simulink model "powertrain_model"  (R2025a)
settings: Solver=ode23tb  StartTime=0.0  StopTime=simlength  FixedStep=tc  MaxStep=tc
values from neighbouring files (symbols this model uses):
  angle_error = angle_error_deg/180*pi    (= 0)    [init_model.m]
  CTRPIFF_CLIP_RELEASE = 0.001    [init_model.m]
  dead_time = dead_time_INV    (= 4.2e-07)    [init_model.m]
  dead_time_INV = 0.42e-6    (= 4.2e-07)    [init_model.m]
  DThs_init = 0    [init_model.m]
  emf_fb_p = 0.2    [init_model.m]
  emf_fb_p_ccaller_1 = emf_fb_p    (= 0.2)    [init_model.m]
  emf_fb_p_ccaller_2 = emf_fb_p    (= 0.2)    [init_model.m]
  emf_p = emf_fb_p*4/10    (= 0.08)    [init_model.m]
  emf_p_ccaller_1 = emf_fb_p_ccaller_1*4/10    (= 0.08)    [init_model.m]
  emf_p_ccaller_2 = emf_fb_p_ccaller_2*4/10    (= 0.08)    [init_model.m]
  fPWM_INV = 25e3    (= 25000)    [init_model.m]
  g0_reference_flt = fcut_reference_flt * ts_inv * 2*pi    (= 0.00100530964915)    [init_model.m]
  g1_reference_flt = 1 - g0_reference_flt    (= 0.998994690351)    [init_model.m]
  id_ref_if_pu = iload_rms_ref*sqrt(2)/ibez    [init_model.m]
  kalman_omega = kw    [init_model.m]
  kalman_theta = kg    [init_model.m]
  kg = K(1)    [init_model.m]
  ki_id = 2    [analysis_cc.m]    (also in init_model.m = 9)
  ki_iq = 9    [init_model.m]
  ki_w = 1    [init_model.m]
  kp_id = 0.15    [analysis_cc.m]    (also in init_model.m = 0.25)
  kp_iq = 0.2    [init_model.m]
  kp_w = 1    [init_model.m]
  kw = K(2)    [init_model.m]
  luenberger_l1 = Klo(1)    [init_model.m]
  luenberger_l2 = Klo(2)    [init_model.m]
  luenberger_l3 = Klo(3)    [init_model.m]
  motorc_m_scale = 2/3*Vdc_bez/ubez    [init_model.m]
  number_of_cells = 100    [init_model.m]
  omega_flt_fcut = 10    [init_model.m]
  omega_flt_g0 = omega_flt_fcut * ts_inv * 2*pi    (= 0.00251327412287)    [init_model.m]
  omega_flt_g1 = 1 - omega_flt_g0    (= 0.997486725877)    [init_model.m]
  omega_ref_if_pu = 1200*2*pi/omega_bez    [init_model.m]
  phase_compensation_omega = 0    [init_model.m]
  pwm_out_lim = 1    [init_model.m]
  Q = 10    [init_model.m]
  q1Kalman = ts_inv^2    (= 1.6e-09)    [init_model.m]
  q2Kalman = ts_inv^1    (= 4e-05)    [init_model.m]
  q3Kalman = 0    [init_model.m]
  rKalman = 1    [init_model.m]
  Tambient = 1    [init_model.m]
  tc = ts_inv/200    (= 2e-07)    [init_model.m]
  time_init = 0.025    [init_model.m]
  torque_ref = 64/ibez*torque_mode    [init_model.m]
  ts_inv = 1/fPWM_INV    (= 4e-05)    [init_model.m]
  tsample = ts_inv    (= 4e-05)    [init_model.m]
  u_flt_g0 = u_flt_fcut * ts_inv * 2*pi    (= 0.904778684234)    [init_model.m]
  u_flt_g1 = 1 - u_flt_g0    (= 0.0952213157661)    [init_model.m]
  Vdc_bez = 400    [init_model.m]
undefined symbols (not defined in the file or in its folder): b, ibez, Jm, Jm_norm, Ld_norm, Lq_norm, Ls_norm, magnitude, omega_bez, psi_bez, psi_m, psi_m_norm, R_RLload, Rload_eq, Rs_norm, tau_bez, weigth
libraries: fl_lib x100, nesl_utility x84, ee_lib x11, cstblocks x4, lithium_ion_cell_lib x1, simulink x1, pmsm_uvw_with_harmonics_lib x1, pmsm_spatial_harmonics_uvw_lib x1, flexshaft_lib x1
(part 1 of 6)
settings Model: SimulationMode=accelerator  Creator=dbagn  LastModifiedBy=dbagn
settings SolverCC: NumberNewtonIterations=3.0  ZeroCrossControl=DisableAll  AlgebraicLoopSolver=TrustRegion  SolverResetMethod=Robust
settings DataIOCC: SaveOutput=off  SignalLogging=off  DSMLogging=off  SaveTime=off  ReturnWorkspaceOutputs=off
settings OptimizationCC: ReuseModelBlockBuffer=off
settings DebuggingCC: UnconnectedInputMsg=warning  UnconnectedOutputMsg=warning  UnconnectedLineMsg=warning
settings ModelReferenceCC: EnableRefExpFcnMdlSchedulingChecks=on
settings SFSimCC: SimUserIncludeDirs=include  SimAnalyzeCustomCode=on
settings SFSimCC: SimCustomHeaderCode=|
  | #include "mavgflt.h"
  | #include "bemf_obsv.h"
  | #include "dqvector_pi.h"
  | #include "dqvector_pi_simulink.h"
  | #include "mavgflt_simulink.h"
  | #include "sv_pwm.h"
  | #include "bemf_obsv_simulink.h"
  | #include "bemf_obsv_load_est.h"
  | #include "bemf_obsv_load_est_simulink.h"
  | #include "sv_pwm_simulink.h"
  | #include "fb_state_machine.h"
  | #include "fb_state_machine_simulink.h"
settings SFSimCC: SimUserSources=|
  | dqvector_pi.c
  | dqvector_pi_simulink.c
  | mavgflt_simulink.c
  | mavgflt.c
  | bemf_obsv_simulink.c
  | bemf_obsv.c
  | bemf_obsv_load_est_simulink.c
  | bemf_obsv_load_est.c
  | sv_pwm.c
  | sv_pwm_simulink.c
  | fb_state_machine.c
  | fb_state_machine_simulink.c
settings RTWCC: GPUComputeCapability=3.5  DLArmComputeVersion=19.05

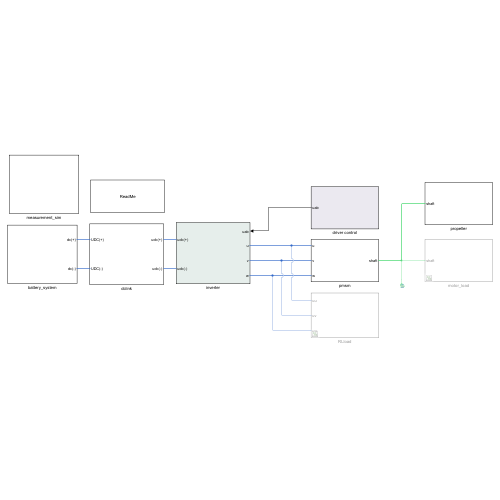
[thumbnail: Simulink's stored preview of the top-level diagram]
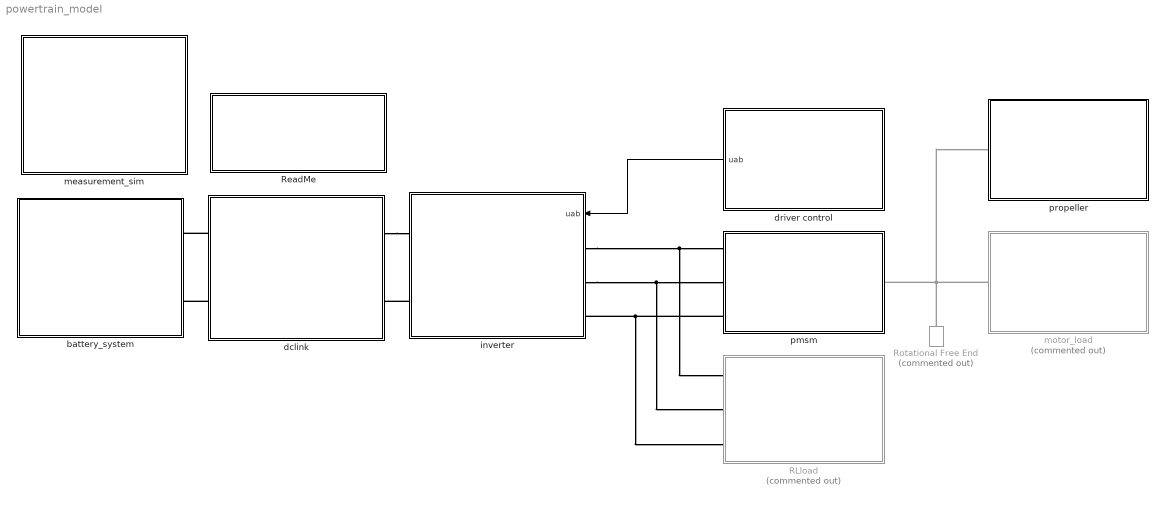
== system powertrain_model ==
  RLload : Subsystem  Commented=on
  ReadMe : Subsystem
      mask Display: disp('ReadMe')
  Rotational Free End : fl_lib/Mechanical/Rotational Elements/Rotational Free End  Commented=on  w_specify=off  w_priority=None  w=0 rad/s  w_nominal_specify=off  w_nominal_value=1  w_nominal_unit=rad/s
  battery_system : Subsystem
  dclink : Subsystem
  driver control : Subsystem
  inverter : Subsystem
  measurement_sim : Subsystem
  motor_load : Subsystem  Commented=on
  pmsm : Subsystem
  propeller : Subsystem
  wires:
  driver control/1(uab) -> inverter/1(uab)
  connections:
  dclink/LConn1 -- battery_system/RConn1
  dclink/LConn2 -- battery_system/RConn2
  inverter/RConn2 -- dclink/RConn2
  dclink/RConn1 -- inverter/RConn1
  motor_load/RConn1 -- pmsm/RConn1 -- propeller/LConn1 -- Rotational Free End/LConn1
  pmsm/LConn3 -- RLload/LConn3 -- inverter/LConn3
  inverter/LConn2 -- RLload/LConn2 -- pmsm/LConn2
  inverter/LConn1 -- RLload/LConn1 -- pmsm/LConn1

== system powertrain_model/RLload ==
  Bus Creator1 : BusCreator  Inputs=3
  Current Sensor : fl_lib/Electrical/Electrical Sensors/Current Sensor
  Current Sensor1 : fl_lib/Electrical/Electrical Sensors/Current Sensor
  Current Sensor2 : fl_lib/Electrical/Electrical Sensors/Current Sensor
  Inductor : ee_lib/Passive/Inductor  l=L_RLload H  enable_L_tol=0  L_tol=20  tol_distribution=1  nSigma=4  r=0 Ohm  g=1e-9 1/Ohm  enable_operating_limits=0  operating_limit_action=2  max_working_current=1 A  power_rating=1 W  i_L_specify=off  i_L_priority=High  i_L=0 A  i_L_nominal_specify=off  i_L_nominal_value=1  i_L_nominal_unit=A
  Inductor1 : ee_lib/Passive/Inductor  l=L_RLload H  enable_L_tol=0  L_tol=20  tol_distribution=1  nSigma=4  r=0 Ohm  g=1e-9 1/Ohm  enable_operating_limits=0  operating_limit_action=2  max_working_current=1 A  power_rating=1 W  i_L_specify=off  i_L_priority=High  i_L=0 A  i_L_nominal_specify=off  i_L_nominal_value=1  i_L_nominal_unit=A
  Inductor2 : ee_lib/Passive/Inductor  l=L_RLload H  enable_L_tol=0  L_tol=20  tol_distribution=1  nSigma=4  r=0 Ohm  g=1e-9 1/Ohm  enable_operating_limits=0  operating_limit_action=2  max_working_current=1 A  power_rating=1 W  i_L_specify=off  i_L_priority=High  i_L=0 A  i_L_nominal_specify=off  i_L_nominal_value=1  i_L_nominal_unit=A
  PS-Simulink Converter1 : nesl_utility/PS-Simulink Converter  PhysicalDomain=network_engine_domain  SubClassName=ps_output  LeftPortType=input  RightPortType=output  PseudoPeriodic=off  Frequencies=[]  VectorFormat=1-D array  Unit=A  AffineConversion=off
  PS-Simulink Converter2 : nesl_utility/PS-Simulink Converter  PhysicalDomain=network_engine_domain  SubClassName=ps_output  LeftPortType=input  RightPortType=output  PseudoPeriodic=off  Frequencies=[]  VectorFormat=1-D array  Unit=A  AffineConversion=off
  PS-Simulink Converter3 : nesl_utility/PS-Simulink Converter  PhysicalDomain=network_engine_domain  SubClassName=ps_output  LeftPortType=input  RightPortType=output  PseudoPeriodic=off  Frequencies=[]  VectorFormat=1-D array  Unit=A  AffineConversion=off
  Resistor : fl_lib/Electrical/Electrical Elements/Resistor  R=R_RLload Ohm  i_specify=off  i_priority=None  i=0 A  i_nominal_specify=off  i_nominal_value=1  i_nominal_unit=A  v_specify=off  v_priority=None  v=0 V  v_nominal_specify=off  v_nominal_value=1  v_nominal_unit=V
  Resistor1 : fl_lib/Electrical/Electrical Elements/Resistor  R=R_RLload Ohm  i_specify=off  i_priority=None  i=0 A  i_nominal_specify=off  i_nominal_value=1  i_nominal_unit=A  v_specify=off  v_priority=None  v=0 V  v_nominal_specify=off  v_nominal_value=1  v_nominal_unit=V
  Resistor2 : fl_lib/Electrical/Electrical Elements/Resistor  R=R_RLload Ohm  i_specify=off  i_priority=None  i=0 A  i_nominal_specify=off  i_nominal_value=1  i_nominal_unit=A  v_specify=off  v_priority=None  v=0 V  v_nominal_specify=off  v_nominal_value=1  v_nominal_unit=V
  iuvw_load : Scope
      settings: SampleTime=tc  ActiveDisplayYMinimum=-116.88009  ActiveDisplayYMaximum=116.86904
  uu : PMIOPort  Side=Left
  uv : PMIOPort  Port=2  Side=Left
  uw : PMIOPort  Port=3  Side=Left
  wires:
  PS-Simulink Converter1/1 -> Bus Creator1/1  "iu_load_sim"
  Bus Creator1/1 -> iuvw_load/1
  PS-Simulink Converter3/1 -> Bus Creator1/3  "iw_load_sim"
  PS-Simulink Converter2/1 -> Bus Creator1/2  "iv_load_sim"
  connections:
  Resistor1/LConn1 -- uv/RConn1
  uu/RConn1 -- Resistor/LConn1
  Resistor2/LConn1 -- uw/RConn1
  Inductor1/LConn1 -- Resistor1/RConn1
  Resistor/RConn1 -- Inductor/LConn1
  Inductor2/LConn1 -- Resistor2/RConn1
  PS-Simulink Converter3/LConn1 -- Current Sensor2/RConn1
  Current Sensor1/RConn1 -- PS-Simulink Converter2/LConn1
  Current Sensor/RConn2 -- Current Sensor2/RConn2 -- Current Sensor1/RConn2
  Current Sensor/RConn1 -- PS-Simulink Converter1/LConn1
  Current Sensor/LConn1 -- Inductor/RConn1
  Inductor2/RConn1 -- Current Sensor2/LConn1
  Inductor1/RConn1 -- Current Sensor1/LConn1

== system powertrain_model/ReadMe ==

== system powertrain_model/battery_system ==
  DC Voltage Source : fl_lib/Electrical/Electrical Sources/DC Voltage Source  Commented=on  v0=Vdc_bez V
  Electrical Reference2 : fl_lib/Electrical/Electrical Elements/Electrical Reference
  Solver Configuration : nesl_utility/Solver Configuration  PhysicalDomain=network_engine_domain  SubClassName=solver  LeftPortType=input  RightPortType=generic  Tones=[]  Harmonics=[]  SimulateNoise=off  Profile=off  UseLocalSampling=off  EnableSwitchedLinearOptims=on  FrequencyDomain=off  UseCCode=off  RelTol=0.001  AbsTol=0.001  MinStep=1e-09  ToWorkspace=off  RevertToSquareIcSolve=off  NumHomotopyIterations=100  PhasorMode=off  PhasorModeNumHarmonics=1  ConsistencySolver=NEWTON_FTOL  IndexReductionMethod=DerivativeReplacement  DoDC=off  ResidualTolerance=1e-09  ConsistencyTolSource=GLOBAL  ConsistencyAbsTol=0.001  ConsistencyRelTol=0.001  ConsistencyTolFactor=0.001  UseLocalSolver=on  LocalSolverChoice=NE_BACKWARD_EULER_ADVANCER  ResolveIndetEquations=on  FunctionEvalNumThread=1  LocalSolverSampleTime=tc  DoFixedCost=on  MaxNonlinIter=5  MaxModeIter=2  ComputeImpulses=off  ImpulseIterations=2  LinearAlgebra=auto  LinearAlgebraNumThread=0  EquationFormulation=NE_TIME_EF  DelaysMemoryBudget=1024  AutomaticFiltering=on  FilteringTimeConstant=0.001  PartitionStorageMethod=AS_NEEDED  PartitionMemoryBudget=1024  PartitionMethod=ROBUST  MultibodyUseLocalSolver=off  MultibodyLocalSolverChoice=ODE1  MultibodyLocalSolverSampleTime=0.001
  battery_system : Subsystem
  dc(+) : PMIOPort  Side=Right
  dc(-) : PMIOPort  Port=2  Side=Right
  connections:
  Solver Configuration/RConn1 -- DC Voltage Source/RConn1 -- Electrical Reference2/LConn1 -- dc(-)/RConn1
  DC Voltage Source/LConn1 -- dc(+)/RConn1 -- battery_system/RConn1

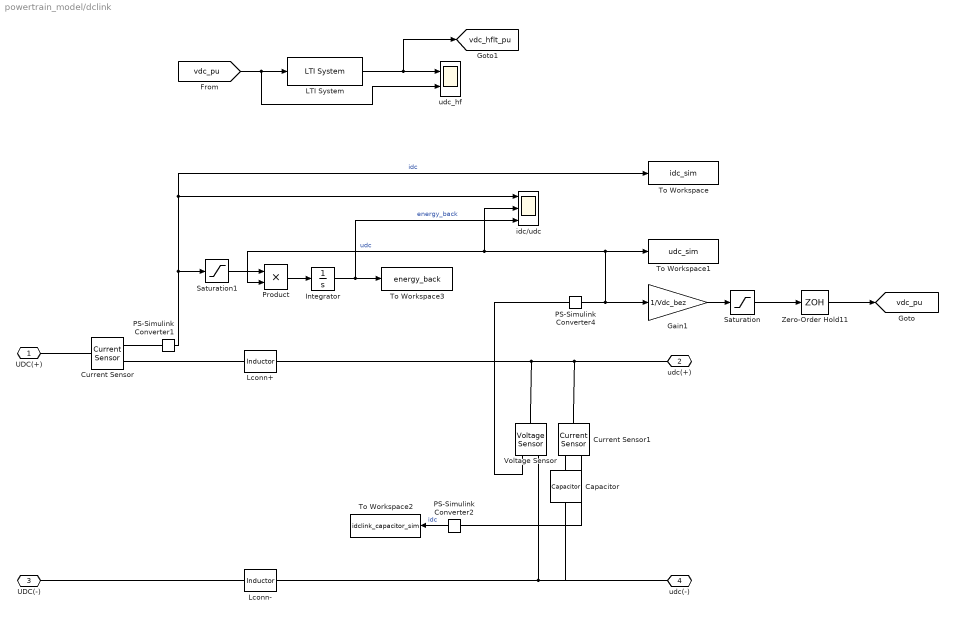
== system powertrain_model/dclink ==
  Capacitor : fl_lib/Electrical/Electrical Elements/Capacitor  c=CFi F  r=1e-3 Ohm  g=0 1/Ohm  i_specify=off  i_priority=None  i=0 A  i_nominal_specify=off  i_nominal_value=1  i_nominal_unit=A  v_specify=off  v_priority=None  v=Vdc_bez V  v_nominal_specify=off  v_nominal_value=1  v_nominal_unit=V  vc_specify=on  vc_priority=High  vc=Vdc V  vc_nominal_specify=off  vc_nominal_value=1  vc_nominal_unit=V
  Current Sensor : fl_lib/Electrical/Electrical Sensors/Current Sensor
  Current Sensor1 : fl_lib/Electrical/Electrical Sensors/Current Sensor
  Gain1 : Gain  Gain=1/Vdc_bez
  Integrator : Integrator
  LTI System : cstblocks/LTI System  sys=hpf2q_d  IC=[]  PadeOrder=0
  Lconn+ : fl_lib/Electrical/Electrical Elements/Inductor  l=0.5e-6 H  r=5e-3 Ohm  g=1e-9 1/Ohm  i_specify=on  i_priority=High  i=0 A  i_nominal_specify=off  i_nominal_value=1  i_nominal_unit=A  v_specify=off  v_priority=None  v=0 V  v_nominal_specify=off  v_nominal_value=1  v_nominal_unit=V  i_L_specify=off  i_L_priority=High  i_L=0 A  i_L_nominal_specify=off  i_L_nominal_value=1  i_L_nominal_unit=A
  Lconn- : fl_lib/Electrical/Electrical Elements/Inductor  l=0.5e-6 H  r=5e-3 Ohm  g=1e-9 1/Ohm  i_specify=on  i_priority=High  i=0 A  i_nominal_specify=off  i_nominal_value=1  i_nominal_unit=A  v_specify=off  v_priority=None  v=0 V  v_nominal_specify=off  v_nominal_value=1  v_nominal_unit=V  i_L_specify=off  i_L_priority=High  i_L=0 A  i_L_nominal_specify=off  i_L_nominal_value=1  i_L_nominal_unit=A
  PS-Simulink Converter1 : nesl_utility/PS-Simulink Converter  PhysicalDomain=network_engine_domain  SubClassName=ps_output  LeftPortType=input  RightPortType=output  PseudoPeriodic=off  Frequencies=[]  VectorFormat=1-D array  Unit=A  AffineConversion=on
  PS-Simulink Converter2 : nesl_utility/PS-Simulink Converter  PhysicalDomain=network_engine_domain  SubClassName=ps_output  LeftPortType=input  RightPortType=output  PseudoPeriodic=off  Frequencies=[]  VectorFormat=1-D array  Unit=A  AffineConversion=on
  PS-Simulink Converter4 : nesl_utility/PS-Simulink Converter  PhysicalDomain=network_engine_domain  SubClassName=ps_output  LeftPortType=input  RightPortType=output  PseudoPeriodic=off  Frequencies=[]  VectorFormat=1-D array  Unit=V  AffineConversion=on
  Product : Product
  Saturation : Saturate  UpperLimit=inf  LowerLimit=0.1
  Saturation1 : Saturate  UpperLimit=0  LowerLimit=-inf
  To Workspace : ToWorkspace  VariableName=idc_sim  SampleTime=tc
      settings: MaxDataPoints=Nc
  To Workspace1 : ToWorkspace  VariableName=udc_sim  SampleTime=tc
      settings: MaxDataPoints=Nc
  To Workspace2 : ToWorkspace  VariableName=idclink_capacitor_sim  SampleTime=tc
      settings: MaxDataPoints=Nc
  To Workspace3 : ToWorkspace  VariableName=energy_back  SampleTime=tc
      settings: MaxDataPoints=Nc
  Voltage Sensor : fl_lib/Electrical/Electrical Sensors/Voltage Sensor
  Zero-Order Hold11 : ZeroOrderHold  SampleTime=ts_inv
  idc/udc : Scope  NumInputPorts=3
      settings: SampleTime=tc  ActiveDisplayYMinimum=-8.28263  ActiveDisplayYMaximum=4.59214
  udc_hf : Scope  NumInputPorts=2
      settings: SampleTime=ts_inv  ActiveDisplayYMinimum=-0.00098  ActiveDisplayYMaximum=0.00078
  UDC(+) : PMIOPort  Side=Left
  udc(+) : PMIOPort  Port=2  Side=Right
  UDC(-) : PMIOPort  Port=3  Side=Left
  udc(-) : PMIOPort  Port=4  Side=Right
  tag scope: vdc_hflt_pu=global, vdc_pu=global
  wires:
  Saturation/1 -> Zero-Order Hold11/1
  PS-Simulink Converter4/1 -> idc/udc/2, Product/2, To Workspace1/1, Gain1/1  "udc"
  Gain1/1 -> Saturation/1
  PS-Simulink Converter1/1 -> Saturation1/1, To Workspace/1, idc/udc/1  "idc"
  PS-Simulink Converter2/1 -> To Workspace2/1  "idc"
  Saturation1/1 -> Product/1
  Product/1 -> Integrator/1
  Integrator/1 -> idc/udc/3, To Workspace3/1  "energy_back"
  LTI System/1 -> [vdc_hflt_pu], udc_hf/1
  [vdc_pu] -> udc_hf/2, LTI System/1
  Zero-Order Hold11/1 -> [vdc_pu]
  connections:
  PS-Simulink Converter4/LConn1 -- Voltage Sensor/RConn1
  Current Sensor1/RConn1 -- PS-Simulink Converter2/LConn1
  PS-Simulink Converter1/LConn1 -- Current Sensor/RConn1
  Current Sensor/RConn2 -- Lconn+/LConn1
  Current Sensor/LConn1 -- UDC(+)/RConn1
  Current Sensor1/RConn2 -- Capacitor/LConn1
  Lconn-/RConn1 -- UDC(-)/RConn1
  Lconn+/RConn1 -- Voltage Sensor/LConn1 -- Current Sensor1/LConn1 -- udc(+)/RConn1
  Voltage Sensor/RConn2 -- Lconn-/LConn1 -- Capacitor/RConn1 -- udc(-)/RConn1

== system powertrain_model/driver control ==
  Mux : Mux  Inputs=2
  Mux1 : Mux  Inputs=2
  Mux2 : Mux  Inputs=2
  Sum1 : Sum  Inputs=+++
  Sum2 : Sum  Inputs=+++
  bemf_observer : Subsystem
  current_ctrl : Subsystem
  i/f references : Subsystem  Commented=on
  id/iq/torque/omega : Scope  NumInputPorts=3
      settings: SampleTime=ts_inv  ActiveDisplayYMinimum=-0.27921550957244479  ActiveDisplayYMaximum=1.2654943086208228  DataLoggingVariableName=ScopeData3
  normalization1 : Gain  Gain=1/tau_bez
  normalization2 : Gain  Gain=1/omega_bez
  speed_loop : Subsystem  Commented=on
  torque_reference_generator : Subsystem
  uab : Outport  VectorParamsAs1DForOutWhenUnconnected=off
  wires:
  Mux/1 -> id/iq/torque/omega/1
  [torque_pmsm] -> normalization1/1
  current_ctrl/1(uab) -> uab/1  "uab"
  Sum2/1 -> current_ctrl/2(iq_ref)  "iq_ref"
  normalization1/1 -> Mux1/1  "torque"
  [iq_inverter_pu] -> Mux/2  "iq_inverter_pu"
  [id_inverter_pu] -> Mux/1  "id_inverter_pu"
  [omega_pmsm] -> normalization2/1  "omega_pmsm"
  normalization2/1 -> Mux1/2  "omega_pmsm"
  Mux1/1 -> id/iq/torque/omega/2
  [omega_pu_hat_flt] -> Mux2/1  "omega_hat_flt"
  [omega_pu_hat] -> Mux2/2  "omega_hat"
  Mux2/1 -> id/iq/torque/omega/3
  Sum1/1 -> current_ctrl/1(id_ref)  "iq_ref"
  i/f references/1(id_if_pu) -> Sum1/2
  torque_reference_generator/1(iq_ref) -> Sum2/3  "torque_ref_pu"
  torque_reference_generator/2(id_ref) -> Sum1/3
  i/f references/2(iq_if_pu) -> Sum2/2
  speed_loop/2(id_ref) -> Sum1/1
  speed_loop/1(iq_ref) -> Sum2/1  "torque_ref_pu"

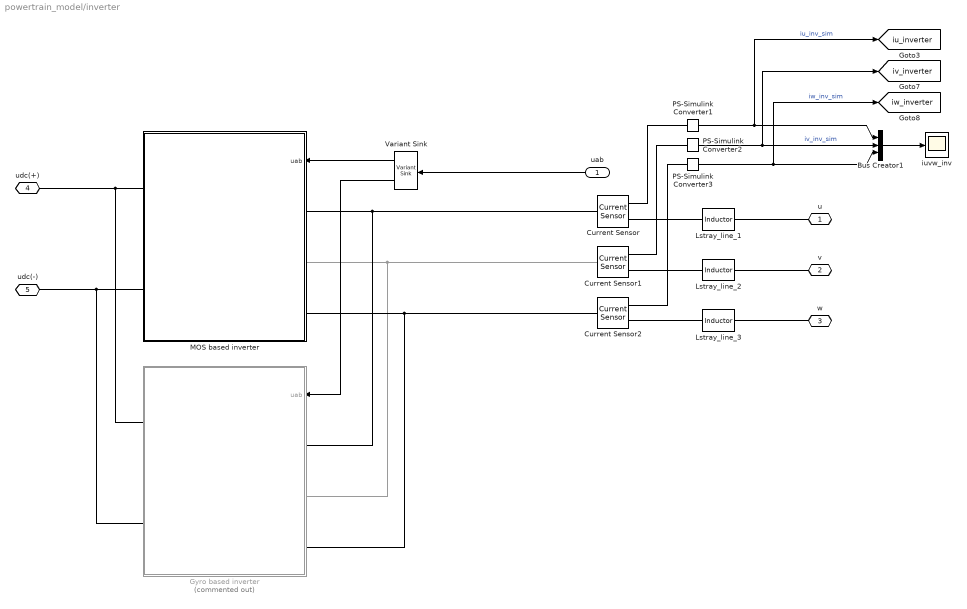
== system powertrain_model/inverter ==
  uab : Inport
  Bus Creator1 : BusCreator  Inputs=3
  Current Sensor : fl_lib/Electrical/Electrical Sensors/Current Sensor
  Current Sensor1 : fl_lib/Electrical/Electrical Sensors/Current Sensor
  Current Sensor2 : fl_lib/Electrical/Electrical Sensors/Current Sensor
  Gyro based inverter : Subsystem  Commented=on
  Lstray_line_1 : ee_lib/Passive/Inductor  l=5e-6 H  enable_L_tol=ee.enum.toleranceApplication.none  L_tol=20  tol_distribution=ee.enum.toleranceDistribution.uniform  nSigma=4  r=0 Ohm  g=1e-9 1/Ohm  enable_operating_limits=ee.enum.enable.no  operating_limit_action=ee.enum.passive.reportOpLim.warn  max_working_current=1 A  power_rating=1 W  i_L_specify=on  i_L_priority=High  i_L=0 A  i_L_nominal_specify=off  i_L_nominal_value=1  i_L_nominal_unit=A
  Lstray_line_2 : ee_lib/Passive/Inductor  l=5e-6 H  enable_L_tol=ee.enum.toleranceApplication.none  L_tol=20  tol_distribution=ee.enum.toleranceDistribution.uniform  nSigma=4  r=0 Ohm  g=1e-9 1/Ohm  enable_operating_limits=ee.enum.enable.no  operating_limit_action=ee.enum.passive.reportOpLim.warn  max_working_current=1 A  power_rating=1 W  i_L_specify=on  i_L_priority=High  i_L=0 A  i_L_nominal_specify=off  i_L_nominal_value=1  i_L_nominal_unit=A
  Lstray_line_3 : ee_lib/Passive/Inductor  l=5e-6 H  enable_L_tol=ee.enum.toleranceApplication.none  L_tol=20  tol_distribution=ee.enum.toleranceDistribution.uniform  nSigma=4  r=0 Ohm  g=1e-9 1/Ohm  enable_operating_limits=ee.enum.enable.no  operating_limit_action=ee.enum.passive.reportOpLim.warn  max_working_current=1 A  power_rating=1 W  i_L_specify=on  i_L_priority=High  i_L=0 A  i_L_nominal_specify=off  i_L_nominal_value=1  i_L_nominal_unit=A
  MOS based inverter : Subsystem
  PS-Simulink Converter1 : nesl_utility/PS-Simulink Converter  PhysicalDomain=network_engine_domain  SubClassName=ps_output  LeftPortType=input  RightPortType=output  PseudoPeriodic=off  Frequencies=[]  VectorFormat=1-D array  Unit=A  AffineConversion=off
  PS-Simulink Converter2 : nesl_utility/PS-Simulink Converter  PhysicalDomain=network_engine_domain  SubClassName=ps_output  LeftPortType=input  RightPortType=output  PseudoPeriodic=off  Frequencies=[]  VectorFormat=1-D array  Unit=A  AffineConversion=off
  PS-Simulink Converter3 : nesl_utility/PS-Simulink Converter  PhysicalDomain=network_engine_domain  SubClassName=ps_output  LeftPortType=input  RightPortType=output  PseudoPeriodic=off  Frequencies=[]  VectorFormat=1-D array  Unit=A  AffineConversion=off
  Variant Sink : VariantSink  VariantControls={use_gyro_model == 0, use_gyro_model == 1}
      settings: AllowZeroVariantControls=on
  iuvw_inv : Scope
      settings: SampleTime=tc  ActiveDisplayYMinimum=-190.27982  ActiveDisplayYMaximum=181.88216
  u : PMIOPort  Side=Left
  v : PMIOPort  Port=2  Side=Left
  w : PMIOPort  Port=3  Side=Left
  udc(+) : PMIOPort  Port=4  Side=Right
  udc(-) : PMIOPort  Port=5  Side=Right
  tag scope: iu_inverter=global, iv_inverter=global, iw_inverter=global
  wires:
  Bus Creator1/1 -> iuvw_inv/1
  PS-Simulink Converter3/1 -> [iw_inverter], Bus Creator1/3  "iw_inv_sim"
  PS-Simulink Converter1/1 -> [iu_inverter], Bus Creator1/1  "iu_inv_sim"
  PS-Simulink Converter2/1 -> [iv_inverter], Bus Creator1/2  "iv_inv_sim"
  uab/1 -> Variant Sink/1
  Variant Sink/1 -> MOS based inverter/1(uab)
  Variant Sink/2 -> Gyro based inverter/1(uab)
  connections:
  Gyro based inverter/LConn2 -- MOS based inverter/LConn2 -- Current Sensor1/LConn1
  MOS based inverter/LConn1 -- Current Sensor/LConn1 -- Gyro based inverter/LConn1
  MOS based inverter/LConn3 -- Current Sensor2/LConn1 -- Gyro based inverter/LConn3
  udc(+)/RConn1 -- Gyro based inverter/RConn1 -- MOS based inverter/RConn1
  udc(-)/RConn1 -- Gyro based inverter/RConn2 -- MOS based inverter/RConn2
  Lstray_line_3/RConn1 -- w/RConn1
  PS-Simulink Converter3/LConn1 -- Current Sensor2/RConn1
  Current Sensor1/RConn1 -- PS-Simulink Converter2/LConn1
  Current Sensor1/RConn2 -- Lstray_line_2/LConn1
  Current Sensor/RConn1 -- PS-Simulink Converter1/LConn1
  Current Sensor/RConn2 -- Lstray_line_1/LConn1
  Lstray_line_2/RConn1 -- v/RConn1
  Current Sensor2/RConn2 -- Lstray_line_3/LConn1
  u/RConn1 -- Lstray_line_1/RConn1

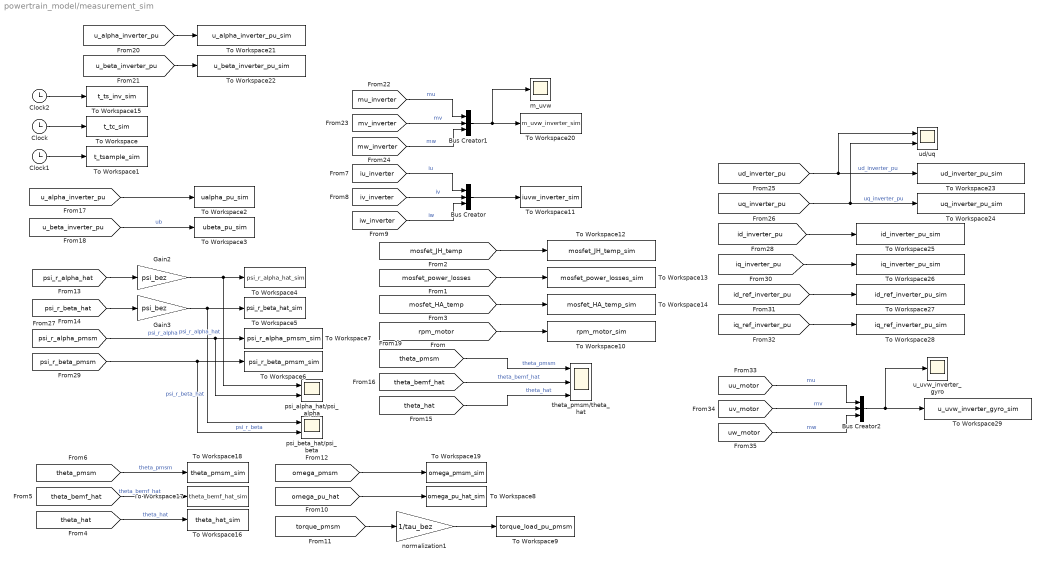
== system powertrain_model/measurement_sim ==
  Bus Creator : BusCreator  Inputs=3
  Bus Creator1 : BusCreator  Inputs=3
  Bus Creator2 : BusCreator  Inputs=3
  Clock : Clock
  Clock1 : Clock
  Clock2 : Clock
  Gain2 : Gain  Gain=psi_bez
  Gain3 : Gain  Gain=psi_bez
  To Workspace : ToWorkspace  VariableName=t_tc_sim  SampleTime=tc
      settings: MaxDataPoints=Nc
  To Workspace1 : ToWorkspace  VariableName=t_tsample_sim  SampleTime=tsample
      settings: MaxDataPoints=Nsample
  To Workspace10 : ToWorkspace  VariableName=rpm_motor_sim  SampleTime=ts_inv
      settings: MaxDataPoints=Ns_inv
  To Workspace11 : ToWorkspace  VariableName=iuvw_inverter_sim  SampleTime=tc
      settings: MaxDataPoints=Nc
  To Workspace12 : ToWorkspace  VariableName=mosfet_JH_temp_sim  SampleTime=tc
      settings: MaxDataPoints=Nc
  To Workspace13 : ToWorkspace  VariableName=mosfet_power_losses_sim  SampleTime=tc
      settings: MaxDataPoints=Nc
  To Workspace14 : ToWorkspace  VariableName=mosfet_HA_temp_sim  SampleTime=tc
      settings: MaxDataPoints=Nc
  To Workspace15 : ToWorkspace  VariableName=t_ts_inv_sim  SampleTime=ts_inv
      settings: MaxDataPoints=Ns_inv
  To Workspace16 : ToWorkspace  VariableName=theta_hat_sim  SampleTime=ts_inv
      settings: MaxDataPoints=Ns_inv
  To Workspace17 : ToWorkspace  VariableName=theta_bemf_hat_sim  SampleTime=ts_inv
      settings: MaxDataPoints=Ns_inv
  To Workspace18 : ToWorkspace  VariableName=theta_pmsm_sim  SampleTime=ts_inv
      settings: MaxDataPoints=Ns_inv
  To Workspace19 : ToWorkspace  VariableName=omega_pmsm_sim  SampleTime=ts_inv
      settings: MaxDataPoints=Ns_inv
  To Workspace2 : ToWorkspace  VariableName=ualpha_pu_sim  SampleTime=ts_inv
      settings: MaxDataPoints=Ns_inv
  To Workspace20 : ToWorkspace  VariableName=m_uvw_inverter_sim  SampleTime=tc
      settings: MaxDataPoints=Nc
  To Workspace21 : ToWorkspace  VariableName=u_alpha_inverter_pu_sim  SampleTime=tc
      settings: MaxDataPoints=Nc
  To Workspace22 : ToWorkspace  VariableName=u_beta_inverter_pu_sim  SampleTime=tc
      settings: MaxDataPoints=Nc
  To Workspace23 : ToWorkspace  VariableName=ud_inverter_pu_sim  SampleTime=tc
      settings: MaxDataPoints=Nc
  To Workspace24 : ToWorkspace  VariableName=uq_inverter_pu_sim  SampleTime=tc
      settings: MaxDataPoints=Nc
  To Workspace25 : ToWorkspace  VariableName=id_inverter_pu_sim  SampleTime=tc
      settings: MaxDataPoints=Nc
  To Workspace26 : ToWorkspace  VariableName=iq_inverter_pu_sim  SampleTime=tc
      settings: MaxDataPoints=Nc
  To Workspace27 : ToWorkspace  VariableName=id_ref_inverter_pu_sim  SampleTime=tc
      settings: MaxDataPoints=Nc
  To Workspace28 : ToWorkspace  VariableName=iq_ref_inverter_pu_sim  SampleTime=tc
      settings: MaxDataPoints=Nc
  To Workspace29 : ToWorkspace  VariableName=u_uvw_inverter_gyro_sim  SampleTime=tc
      settings: MaxDataPoints=Nc
  To Workspace3 : ToWorkspace  VariableName=ubeta_pu_sim  SampleTime=ts_inv
      settings: MaxDataPoints=Ns_inv
  To Workspace4 : ToWorkspace  VariableName=psi_r_alpha_hat_sim  SampleTime=ts_inv
      settings: MaxDataPoints=Ns_inv
  To Workspace5 : ToWorkspace  VariableName=psi_r_beta_hat_sim  SampleTime=ts_inv
      settings: MaxDataPoints=Ns_inv
  To Workspace6 : ToWorkspace  VariableName=psi_r_beta_pmsm_sim  SampleTime=ts_inv
      settings: MaxDataPoints=Ns_inv
  To Workspace7 : ToWorkspace  VariableName=psi_r_alpha_pmsm_sim  SampleTime=ts_inv
      settings: MaxDataPoints=Ns_inv
  To Workspace8 : ToWorkspace  VariableName=omega_pu_hat_sim  SampleTime=ts_inv
      settings: MaxDataPoints=Ns_inv
  To Workspace9 : ToWorkspace  VariableName=torque_load_pu_pmsm  SampleTime=ts_inv
      settings: MaxDataPoints=Ns_inv
  m_uvw : Scope
      settings: SampleTime=ts_inv  ActiveDisplayYMinimum=0.41574  ActiveDisplayYMaximum=0.59549  DataLoggingVariableName=ScopeData2
  normalization1 : Gain  Gain=1/tau_bez
  psi_alpha_hat/psi_alpha : Scope  NumInputPorts=2
      settings: SampleTime=ts_inv  ActiveDisplayYMinimum=-0.030406717651633802  ActiveDisplayYMaximum=0.030440385944099833  DataLoggingVariableName=ScopeData2
  psi_beta_hat/psi_beta : Scope  NumInputPorts=2
      settings: SampleTime=ts_inv  ActiveDisplayYMinimum=-0.02688  ActiveDisplayYMaximum=0.02688  DataLoggingVariableName=ScopeData3
  theta_pmsm/theta_hat : Scope  NumInputPorts=3
      settings: SampleTime=tc  ActiveDisplayYMinimum=-3.9269753976279205  ActiveDisplayYMaximum=3.9268824807461784
  u_uvw_inverter_gyro : Scope
      settings: SampleTime=ts_inv  ActiveDisplayYMinimum=-1.24968  ActiveDisplayYMaximum=1.24993
  ud/uq : Scope  NumInputPorts=2
      settings: SampleTime=ts_inv  ActiveDisplayYMinimum=-0.81271  ActiveDisplayYMaximum=0.72345
  wires:
  [psi_r_beta_hat] -> Gain3/1
  [psi_r_alpha_hat] -> Gain2/1
  [u_alpha_inverter_pu] -> To Workspace2/1
  [psi_r_alpha_pmsm] -> psi_alpha_hat/psi_alpha/2, To Workspace7/1  "psi_r_alpha"
  Clock1/1 -> To Workspace1/1
  Clock/1 -> To Workspace/1
  [u_beta_inverter_pu] -> To Workspace3/1  "ub"
  [psi_r_beta_pmsm] -> To Workspace6/1, psi_beta_hat/psi_beta/2  "psi_r_beta"
  [rpm_motor] -> To Workspace10/1
  [iv_inverter] -> Bus Creator/2  "iv"
  [iw_inverter] -> Bus Creator/3  "iw"
  [iu_inverter] -> Bus Creator/1  "iu"
  Bus Creator/1 -> To Workspace11/1
  [mosfet_JH_temp] -> To Workspace12/1
  [mosfet_power_losses] -> To Workspace13/1
  [mosfet_HA_temp] -> To Workspace14/1
  Clock2/1 -> To Workspace15/1
  [theta_bemf_hat] -> To Workspace17/1  "theta_bemf_hat"
  [theta_hat] -> To Workspace16/1  "theta_hat"
  [theta_pmsm] -> To Workspace18/1  "theta_pmsm"
  Gain2/1 -> To Workspace4/1, psi_alpha_hat/psi_alpha/1  "psi_r_alpha_hat"
  Gain3/1 -> psi_beta_hat/psi_beta/1, To Workspace5/1  "psi_r_beta_hat"
  [omega_pmsm] -> To Workspace19/1
  [omega_pu_hat] -> To Workspace8/1
  normalization1/1 -> To Workspace9/1
  [torque_pmsm] -> normalization1/1
  [theta_hat] -> theta_pmsm/theta_hat/3  "theta_hat"
  [theta_bemf_hat] -> theta_pmsm/theta_hat/2  "theta_bemf_hat"
  [theta_pmsm] -> theta_pmsm/theta_hat/1  "theta_pmsm"
  Bus Creator1/1 -> m_uvw/1, To Workspace20/1
  [mu_inverter] -> Bus Creator1/1  "mu"
  [mw_inverter] -> Bus Creator1/3  "mw"
  [mv_inverter] -> Bus Creator1/2  "mv"
  [u_beta_inverter_pu] -> To Workspace22/1
  [u_alpha_inverter_pu] -> To Workspace21/1
  [ud_inverter_pu] -> To Workspace23/1, ud/uq/1  "ud_inverter_pu"
  [uq_inverter_pu] -> ud/uq/2, To Workspace24/1  "uq_inverter_pu"
  [id_inverter_pu] -> To Workspace25/1
  [iq_inverter_pu] -> To Workspace26/1
  [id_ref_inverter_pu] -> To Workspace27/1
  [iq_ref_inverter_pu] -> To Workspace28/1
  [uu_motor] -> Bus Creator2/1  "mu"
  Bus Creator2/1 -> u_uvw_inverter_gyro/1, To Workspace29/1
  [uw_motor] -> Bus Creator2/3  "mw"
  [uv_motor] -> Bus Creator2/2  "mv"

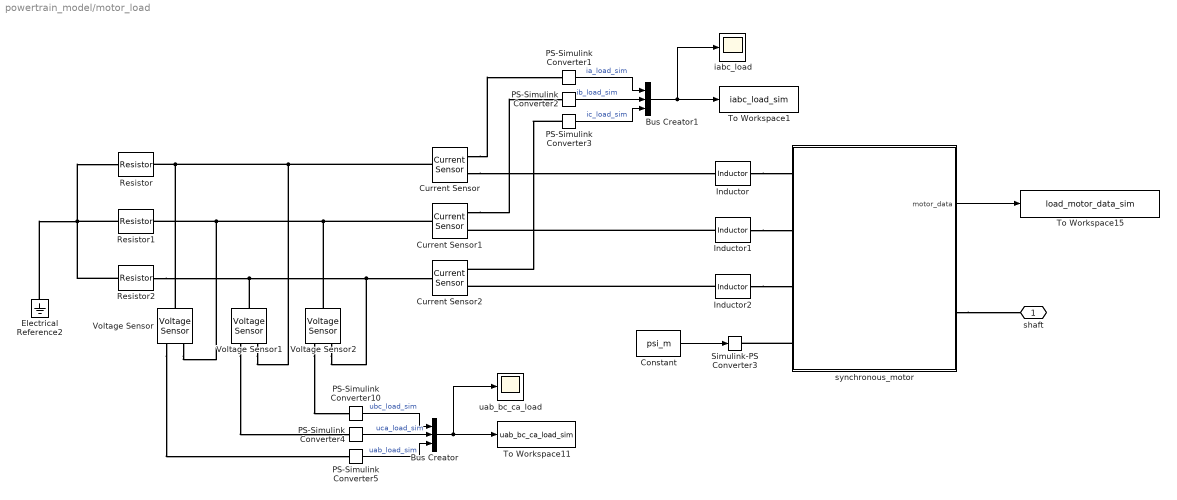
== system powertrain_model/motor_load ==
  Bus Creator : BusCreator  Inputs=3
  Bus Creator1 : BusCreator  Inputs=3
  Constant : Constant  Value=psi_m
  Current Sensor : fl_lib/Electrical/Electrical Sensors/Current Sensor
  Current Sensor1 : fl_lib/Electrical/Electrical Sensors/Current Sensor
  Current Sensor2 : fl_lib/Electrical/Electrical Sensors/Current Sensor
  Electrical Reference2 : fl_lib/Electrical/Electrical Elements/Electrical Reference
  Inductor : ee_lib/Passive/Inductor  l=Lload_eq H  enable_L_tol=0  L_tol=20  tol_distribution=1  nSigma=4  r=0 Ohm  g=1e-9 1/Ohm  enable_operating_limits=0  operating_limit_action=2  max_working_current=1 A  power_rating=1 W  i_L_specify=off  i_L_priority=High  i_L=0 A  i_L_nominal_specify=off  i_L_nominal_value=1  i_L_nominal_unit=A
  Inductor1 : ee_lib/Passive/Inductor  l=Lload_eq H  enable_L_tol=0  L_tol=20  tol_distribution=1  nSigma=4  r=0 Ohm  g=1e-9 1/Ohm  enable_operating_limits=0  operating_limit_action=2  max_working_current=1 A  power_rating=1 W  i_L_specify=off  i_L_priority=High  i_L=0 A  i_L_nominal_specify=off  i_L_nominal_value=1  i_L_nominal_unit=A
  Inductor2 : ee_lib/Passive/Inductor  l=Lload_eq H  enable_L_tol=0  L_tol=20  tol_distribution=1  nSigma=4  r=0 Ohm  g=1e-9 1/Ohm  enable_operating_limits=0  operating_limit_action=2  max_working_current=1 A  power_rating=1 W  i_L_specify=off  i_L_priority=High  i_L=0 A  i_L_nominal_specify=off  i_L_nominal_value=1  i_L_nominal_unit=A
  PS-Simulink Converter1 : nesl_utility/PS-Simulink Converter  PhysicalDomain=network_engine_domain  SubClassName=ps_output  LeftPortType=input  RightPortType=output  PseudoPeriodic=off  Frequencies=[]  VectorFormat=1-D array  Unit=A  AffineConversion=on
  PS-Simulink Converter10 : nesl_utility/PS-Simulink Converter  PhysicalDomain=network_engine_domain  SubClassName=ps_output  LeftPortType=input  RightPortType=output  PseudoPeriodic=off  Frequencies=[]  VectorFormat=1-D array  Unit=V  AffineConversion=on
  PS-Simulink Converter2 : nesl_utility/PS-Simulink Converter  PhysicalDomain=network_engine_domain  SubClassName=ps_output  LeftPortType=input  RightPortType=output  PseudoPeriodic=off  Frequencies=[]  VectorFormat=1-D array  Unit=A  AffineConversion=on
  PS-Simulink Converter3 : nesl_utility/PS-Simulink Converter  PhysicalDomain=network_engine_domain  SubClassName=ps_output  LeftPortType=input  RightPortType=output  PseudoPeriodic=off  Frequencies=[]  VectorFormat=1-D array  Unit=A  AffineConversion=on
  PS-Simulink Converter4 : nesl_utility/PS-Simulink Converter  PhysicalDomain=network_engine_domain  SubClassName=ps_output  LeftPortType=input  RightPortType=output  PseudoPeriodic=off  Frequencies=[]  VectorFormat=1-D array  Unit=V  AffineConversion=on
  PS-Simulink Converter5 : nesl_utility/PS-Simulink Converter  PhysicalDomain=network_engine_domain  SubClassName=ps_output  LeftPortType=input  RightPortType=output  PseudoPeriodic=off  Frequencies=[]  VectorFormat=1-D array  Unit=V  AffineConversion=on
  Resistor : fl_lib/Electrical/Electrical Elements/Resistor  R=Rload_eq Ohm  i_specify=off  i_priority=None  i=0 A  i_nominal_specify=off  i_nominal_value=1  i_nominal_unit=A  v_specify=off  v_priority=None  v=0 V  v_nominal_specify=off  v_nominal_value=1  v_nominal_unit=V
  Resistor1 : fl_lib/Electrical/Electrical Elements/Resistor  R=Rload_eq Ohm  i_specify=off  i_priority=None  i=0 A  i_nominal_specify=off  i_nominal_value=1  i_nominal_unit=A  v_specify=off  v_priority=None  v=0 V  v_nominal_specify=off  v_nominal_value=1  v_nominal_unit=V
  Resistor2 : fl_lib/Electrical/Electrical Elements/Resistor  R=Rload_eq Ohm  i_specify=off  i_priority=None  i=0 A  i_nominal_specify=off  i_nominal_value=1  i_nominal_unit=A  v_specify=off  v_priority=None  v=0 V  v_nominal_specify=off  v_nominal_value=1  v_nominal_unit=V
  Simulink-PS Converter3 : nesl_utility/Simulink-PS Converter  PhysicalDomain=network_engine_domain  SubClassName=ps_input  LeftPortType=input  RightPortType=output  PseudoPeriodic=off  Frequencies=[]  NoiseDistribution=none  NoiseParameters=[]  Unit=V*s  AffineConversion=on  FilteringAndDerivatives=provide  SimscapeFilterOrder=1  InputFilterTimeConstant=0.001  UdotUserProvided=0
  To Workspace1 : ToWorkspace  VariableName=iabc_load_sim  SampleTime=tc
      settings: MaxDataPoints=Nc
  To Workspace11 : ToWorkspace  VariableName=uab_bc_ca_load_sim  SampleTime=tc
      settings: MaxDataPoints=Nc
  To Workspace15 : ToWorkspace  VariableName=load_motor_data_sim  SampleTime=tsample
      settings: MaxDataPoints=Nsample
  Voltage Sensor : fl_lib/Electrical/Electrical Sensors/Voltage Sensor
  Voltage Sensor1 : fl_lib/Electrical/Electrical Sensors/Voltage Sensor
  Voltage Sensor2 : fl_lib/Electrical/Electrical Sensors/Voltage Sensor
  iabc_load : Scope
      settings: DataLoggingVariableName=ScopeData2
  synchronous_motor : Subsystem
  uab_bc_ca_load : Scope
  shaft : PMIOPort  Side=Right
  wires:
  Constant/1 -> Simulink-PS Converter3/1
  synchronous_motor/1(motor_data) -> To Workspace15/1
  Bus Creator/1 -> uab_bc_ca_load/1, To Workspace11/1
  PS-Simulink Converter4/1 -> Bus Creator/2  "uca_load_sim"
  PS-Simulink Converter10/1 -> Bus Creator/1  "ubc_load_sim"
  PS-Simulink Converter5/1 -> Bus Creator/3  "uab_load_sim"
  PS-Simulink Converter3/1 -> Bus Creator1/3  "ic_load_sim"
  PS-Simulink Converter1/1 -> Bus Creator1/1  "ia_load_sim"
  PS-Simulink Converter2/1 -> Bus Creator1/2  "ib_load_sim"
  Bus Creator1/1 -> iabc_load/1, To Workspace1/1
  connections:
  synchronous_motor/LConn4 -- Simulink-PS Converter3/RConn1
  Inductor/RConn1 -- synchronous_motor/LConn1
  Inductor2/RConn1 -- synchronous_motor/LConn3
  Inductor1/RConn1 -- synchronous_motor/LConn2
  Electrical Reference2/LConn1 -- Resistor2/LConn1 -- Resistor1/LConn1 -- Resistor/LConn1
  synchronous_motor/RConn1 -- shaft/RConn1
  Current Sensor/LConn1 -- Voltage Sensor1/RConn2 -- Voltage Sensor/LConn1 -- Resistor/RConn1
  Current Sensor1/LConn1 -- Voltage Sensor2/LConn1 -- Resistor1/RConn1 -- Voltage Sensor/RConn2
  Voltage Sensor1/LConn1 -- Resistor2/RConn1 -- Voltage Sensor2/RConn2 -- Current Sensor2/LConn1
  Inductor2/LConn1 -- Current Sensor2/RConn2
  Inductor1/LConn1 -- Current Sensor1/RConn2
  Current Sensor/RConn2 -- Inductor/LConn1
  Voltage Sensor2/RConn1 -- PS-Simulink Converter10/LConn1
  Current Sensor/RConn1 -- PS-Simulink Converter1/LConn1
  Current Sensor1/RConn1 -- PS-Simulink Converter2/LConn1
  PS-Simulink Converter3/LConn1 -- Current Sensor2/RConn1
  Voltage Sensor1/RConn1 -- PS-Simulink Converter4/LConn1
  Voltage Sensor/RConn1 -- PS-Simulink Converter5/LConn1

== system powertrain_model/pmsm ==
  Constant : Constant  Value=psi_m
  Selector : Selector  InputPortWidth=19  IndexOptions=Index vector (dialog)  Indices=16  OutputSizes=1
  Simulink-PS Converter3 : nesl_utility/Simulink-PS Converter  PhysicalDomain=network_engine_domain  SubClassName=ps_input  LeftPortType=input  RightPortType=output  PseudoPeriodic=off  Frequencies=[]  NoiseDistribution=none  NoiseParameters=[]  Unit=V*s  AffineConversion=on  FilteringAndDerivatives=provide  SimscapeFilterOrder=1  InputFilterTimeConstant=0.001  UdotUserProvided=0
  synchronous_motor : Subsystem
  u : PMIOPort  Side=Left
  v : PMIOPort  Port=2  Side=Left
  w : PMIOPort  Port=3  Side=Left
  shaft : PMIOPort  Port=4  Side=Right
  tag scope: rpm_motor=global
  wires:
  synchronous_motor/1(motor_data) -> Selector/1
  Constant/1 -> Simulink-PS Converter3/1
  Selector/1 -> [rpm_motor]
  connections:
  synchronous_motor/LConn3 -- w/RConn1
  synchronous_motor/RConn1 -- shaft/RConn1
  Simulink-PS Converter3/RConn1 -- synchronous_motor/LConn4
  synchronous_motor/LConn1 -- u/RConn1
  synchronous_motor/LConn2 -- v/RConn1

== system powertrain_model/propeller ==
  Gain : Gain  Gain=1/tau_bez
  Ideal Rotational Motion Sensor : fl_lib/Mechanical/Mechanical Sensors/Ideal Rotational Motion Sensor  reference=foundation.enum.MeasurementReference.difference  acceleration_port=false  velocity_port=true  position_port=true  wrap_angle=true  offset=0 rad
  Ideal Torque Sensor : fl_lib/Mechanical/Mechanical Sensors/Ideal Torque Sensor
  Ideal Torque Source : fl_lib/Mechanical/Mechanical Sources/Ideal Torque Source
  Inertia : fl_lib/Mechanical/Rotational Elements/Inertia  inertia=0.02 kg*m^2  num_ports=foundation.enum.numPorts2.one  w_specify=off  w_priority=High  w=0 rad/s  w_nominal_specify=off  w_nominal_value=1  w_nominal_unit=rad/s  t_specify=off  t_priority=None  t=0 N*m  t_nominal_specify=off  t_nominal_value=1  t_nominal_unit=N*m
  Mechanical Rotational Reference : fl_lib/Mechanical/Rotational Elements/Mechanical Rotational Reference
  Mechanical Rotational Reference1 : fl_lib/Mechanical/Rotational Elements/Mechanical Rotational Reference
  PS Add : fl_lib/Physical Signals/Functions/PS Add
  PS Gain : fl_lib/Physical Signals/Functions/PS Gain  gain=-1
  PS Gain1 : fl_lib/Physical Signals/Functions/PS Gain  gain=0
  PS Gain2 : fl_lib/Physical Signals/Functions/PS Gain  gain=2
  PS Lookup Table (1D) : fl_lib/Physical Signals/Lookup Tables/PS Lookup Table (1D)  x=n rpm  f=torque N*m  interp_method=simscape.enum.interpolation.linear  extrap_method=simscape.enum.extrapolation.linear
  PS Lookup Table (1D)1 : fl_lib/Physical Signals/Lookup Tables/PS Lookup Table (1D)  x=n rpm  f=thrust g  interp_method=simscape.enum.interpolation.linear  extrap_method=simscape.enum.extrapolation.linear
  PS Math Function : fl_lib/Physical Signals/Functions/PS Math Function  fcn_choice=foundation.enum.math_function.cos  v=1
  PS Product : fl_lib/Physical Signals/Functions/PS Product
  PS-Simulink Converter : nesl_utility/PS-Simulink Converter  PhysicalDomain=network_engine_domain  SubClassName=ps_output  LeftPortType=input  RightPortType=output  PseudoPeriodic=off  Frequencies=[]  VectorFormat=1-D array  Unit=kg  AffineConversion=off
  PS-Simulink Converter1 : nesl_utility/PS-Simulink Converter  PhysicalDomain=network_engine_domain  SubClassName=ps_output  LeftPortType=input  RightPortType=output  PseudoPeriodic=off  Frequencies=[]  VectorFormat=1-D array  Unit=N*m  AffineConversion=off
  PS-Simulink Converter2 : nesl_utility/PS-Simulink Converter  PhysicalDomain=network_engine_domain  SubClassName=ps_output  LeftPortType=input  RightPortType=output  PseudoPeriodic=off  Frequencies=[]  VectorFormat=1-D array  Unit=N*m  AffineConversion=off
  Subsystem : Subsystem
      mask Display: disp('flexible shaft')
  To Workspace1 : ToWorkspace  VariableName=torque_sim  SampleTime=tc
      settings: MaxDataPoints=Nc
  To Workspace12 : ToWorkspace  VariableName=thrust_sim  SampleTime=tc
      settings: MaxDataPoints=Nc
  shaft : PMIOPort  Side=Left
  tag scope: torque_load_pu=global
  wires:
  PS-Simulink Converter/1 -> To Workspace12/1
  PS-Simulink Converter1/1 -> To Workspace1/1
  PS-Simulink Converter2/1 -> Gain/1
  Gain/1 -> [torque_load_pu]
  connections:
  Ideal Torque Source/LConn1 -- Inertia/LConn1 -- Ideal Torque Sensor/RConn1 -- Ideal Rotational Motion Sensor/LConn1
  Mechanical Rotational Reference1/LConn1 -- Ideal Torque Source/RConn2
  Ideal Rotational Motion Sensor/RConn1 -- Mechanical Rotational Reference/LConn1
  PS Lookup Table (1D)/LConn1 -- PS Lookup Table (1D)1/LConn1 -- Ideal Rotational Motion Sensor/RConn2
  PS-Simulink Converter/LConn1 -- PS Lookup Table (1D)1/RConn1
  PS Lookup Table (1D)/RConn1 -- PS Product/LConn1 -- PS Gain/LConn1 -- PS-Simulink Converter1/LConn1
  Subsystem/LConn1 -- shaft/RConn1
  PS Gain2/RConn1 -- PS Math Function/LConn1
  PS Gain/RConn1 -- PS Add/LConn1
  PS Add/RConn1 -- Ideal Torque Source/RConn1
  PS Gain1/RConn1 -- PS Add/LConn2
  PS Product/RConn1 -- PS Gain1/LConn1
  PS Math Function/RConn1 -- PS Product/LConn2
  Ideal Rotational Motion Sensor/RConn3 -- PS Gain2/LConn1
  Ideal Torque Sensor/RConn2 -- PS-Simulink Converter2/LConn1
  Ideal Torque Sensor/LConn1 -- Subsystem/RConn1

== system powertrain_model/battery_system/battery_system ==
  Electrical Reference1 : fl_lib/Electrical/Electrical Elements/Electrical Reference
  LithiumIonBattery : Subsystem
  Uout+ : PMIOPort  Side=Right
  connections:
  LithiumIonBattery/RConn2 -- Electrical Reference1/LConn1
  LithiumIonBattery/RConn1 -- Uout+/RConn1

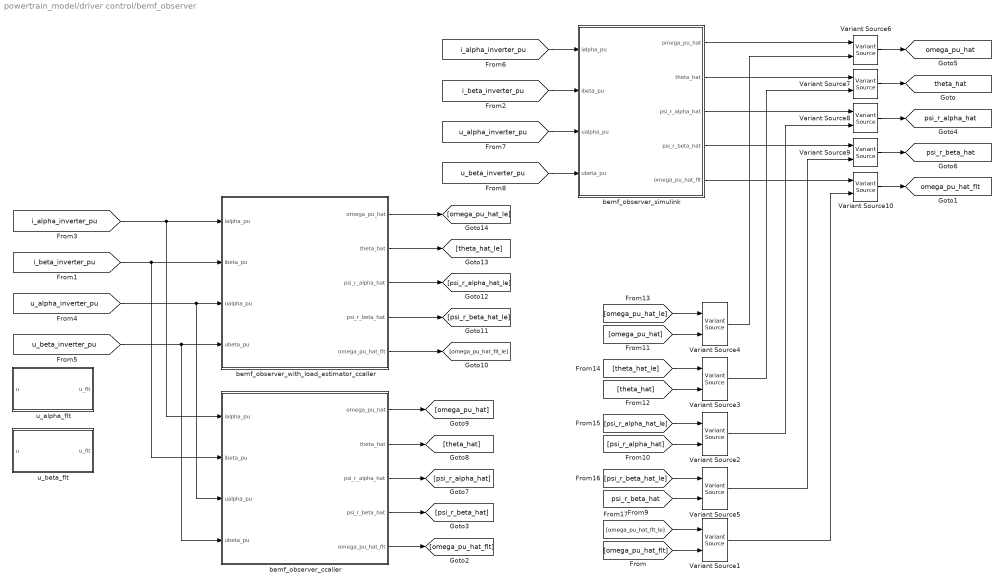
== system powertrain_model/driver control/bemf_observer ==
  Variant Source{1..10} (10 alike) : VariantSource  ShowConditionOnBlock=on
      Variant Source1 settings: AllowZeroVariantControls=on
  bemf_observer_ccaller : Subsystem
  bemf_observer_simulink : Subsystem
  bemf_observer_with_load_estimator_ccaller : Subsystem
  u_alpha_flt : Subsystem
  u_beta_flt : Subsystem
  tag scope: omega_pu_hat=global, omega_pu_hat_flt=global, psi_r_alpha_hat=global, psi_r_beta_hat=global, theta_hat=global
  wires:
  Variant Source6/1 -> [omega_pu_hat]
  [i_alpha_inverter_pu] -> bemf_observer_simulink/1(ialpha_pu)
  [i_beta_inverter_pu] -> bemf_observer_simulink/2(ibeta_pu)
  [u_alpha_inverter_pu] -> bemf_observer_simulink/3(ualpha_pu)
  [u_beta_inverter_pu] -> bemf_observer_simulink/4(ubeta_pu)
  bemf_observer_simulink/1(omega_pu_hat) -> Variant Source6/1
  bemf_observer_simulink/5(omega_pu_hat_flt) -> Variant Source10/1
  bemf_observer_simulink/4(psi_r_beta_hat) -> Variant Source9/1
  bemf_observer_simulink/3(psi_r_alpha_hat) -> Variant Source8/1
  bemf_observer_simulink/2(theta_hat) -> Variant Source7/1
  Variant Source7/1 -> [theta_hat]
  Variant Source8/1 -> [psi_r_alpha_hat]
  Variant Source9/1 -> [psi_r_beta_hat]
  Variant Source10/1 -> [omega_pu_hat_flt]
  [u_alpha_inverter_pu] -> bemf_observer_ccaller/3(ualpha_pu), bemf_observer_with_load_estimator_ccaller/3(ualpha_pu)
  [u_beta_inverter_pu] -> bemf_observer_ccaller/4(ubeta_pu), bemf_observer_with_load_estimator_ccaller/4(ubeta_pu)
  [i_beta_inverter_pu] -> bemf_observer_ccaller/2(ibeta_pu), bemf_observer_with_load_estimator_ccaller/2(ibeta_pu)
  [i_alpha_inverter_pu] -> bemf_observer_ccaller/1(ialpha_pu), bemf_observer_with_load_estimator_ccaller/1(ialpha_pu)
  bemf_observer_ccaller/5(omega_pu_hat_flt) -> [omega_pu_hat_flt]
  [omega_pu_hat_flt] -> Variant Source1/2
  bemf_observer_ccaller/4(psi_r_beta_hat) -> [psi_r_beta_hat]
  bemf_observer_ccaller/1(omega_pu_hat) -> [omega_pu_hat]
  bemf_observer_ccaller/2(theta_hat) -> [theta_hat]
  bemf_observer_ccaller/3(psi_r_alpha_hat) -> [psi_r_alpha_hat]
  [psi_r_beta_hat] -> Variant Source5/2
  [psi_r_alpha_hat] -> Variant Source2/2
  [omega_pu_hat] -> Variant Source4/2
  [theta_hat] -> Variant Source3/2
  bemf_observer_with_load_estimator_ccaller/1(omega_pu_hat) -> [omega_pu_hat_le]
  bemf_observer_with_load_estimator_ccaller/5(omega_pu_hat_flt) -> [omega_pu_hat_flt_le]
  bemf_observer_with_load_estimator_ccaller/4(psi_r_beta_hat) -> [psi_r_beta_hat_le]
  bemf_observer_with_load_estimator_ccaller/3(psi_r_alpha_hat) -> [psi_r_alpha_hat_le]
  bemf_observer_with_load_estimator_ccaller/2(theta_hat) -> [theta_hat_le]
  [omega_pu_hat_le] -> Variant Source4/1
  [theta_hat_le] -> Variant Source3/1
  [psi_r_alpha_hat_le] -> Variant Source2/1
  [psi_r_beta_hat_le] -> Variant Source5/1
  [omega_pu_hat_flt_le] -> Variant Source1/1
  Variant Source4/1 -> Variant Source6/2
  Variant Source3/1 -> Variant Source7/2
  Variant Source2/1 -> Variant Source8/2
  Variant Source5/1 -> Variant Source9/2
  Variant Source1/1 -> Variant Source10/2

== system powertrain_model/driver control/current_ctrl ==
  id_ref : Inport
  iq_ref : Inport  Port=2
  Bus Creator1 : BusCreator  Inputs=2
  Unit Delay{1..4} (4 alike) : UnitDelay  SampleTime=ts_inv  HasFrameUpgradeWarning=on
  current_transformation : Subsystem
  dq2alphabeta : MATLAB Function  TreatAsAtomicUnit=on  SystemSampleTime=ts_inv
  dq2alphabeta1 : MATLAB Function  TreatAsAtomicUnit=on  SystemSampleTime=ts_inv
  rotor_phase_selection : Subsystem
  sample_hold_normalization : Subsystem
  vector_current_ctrl : Subsystem
  uab : Outport  VectorParamsAs1DForOutWhenUnconnected=off
  tag scope: i_alpha_inverter_ref_pu=global, i_beta_inverter_ref_pu=global, u_alpha_inverter_pu=global, u_beta_inverter_pu=global
  wires:
  dq2alphabeta/2(beta) -> Unit Delay2/1  "ub"
  Bus Creator1/1 -> uab/1
  sample_hold_normalization/2(iv_pu) -> current_transformation/2(v)
  sample_hold_normalization/1(iu_pu) -> current_transformation/1(u)
  sample_hold_normalization/3(iw_pu) -> current_transformation/3(w)
  vector_current_ctrl/2(uq) -> dq2alphabeta/2(q)
  vector_current_ctrl/1(ud) -> dq2alphabeta/1(d)
  dq2alphabeta/1(alpha) -> Unit Delay1/1  "ua"
  [iv_inverter] -> sample_hold_normalization/2(iv)  "iv"
  [iu_inverter] -> sample_hold_normalization/1(iu)  "iu"
  [iw_inverter] -> sample_hold_normalization/3(iw)  "iw"
  iq_ref/1 -> dq2alphabeta1/2(q), vector_current_ctrl/1(iq_ref)
  id_ref/1 -> dq2alphabeta1/1(d), vector_current_ctrl/2(id_ref)
  Unit Delay1/1 -> [u_alpha_inverter_pu], Bus Creator1/1  "ua"
  Unit Delay2/1 -> [u_beta_inverter_pu], Bus Creator1/2  "ub"
  rotor_phase_selection/1(theta_ctrl) -> current_transformation/4(phase), dq2alphabeta/3(phase), dq2alphabeta1/3(phase)
  dq2alphabeta1/1(alpha) -> Unit Delay3/1  "ia_ref"
  dq2alphabeta1/2(beta) -> Unit Delay4/1  "ib_ref"
  Unit Delay3/1 -> [i_alpha_inverter_ref_pu]  "ia_ref"
  Unit Delay4/1 -> [i_beta_inverter_ref_pu]  "ib_ref"

== system powertrain_model/driver control/i//f references ==
  Constant : Constant  Value=0
  Constant1 : Constant  Value=omega_ref_if_pu
  Constant2 : Constant  Value=id_ref_if_pu
  Sum1 : Sum  SaturateOnIntegerOverflow=on
  Unit Delay4 : UnitDelay  SampleTime=ts_inv  HasFrameUpgradeWarning=on
  bounder2 : MATLAB Function  TreatAsAtomicUnit=on  SystemSampleTime=ts_inv
  filter_pt1 : Subsystem
  filter_pt2 : Subsystem
  id_ref : Step  Time=time_init  After=id_ref_if_pu  SampleTime=0
  kp : Gain  Gain=omega_bez*ts_inv  SaturateOnIntegerOverflow=on  OutDataTypeStr=Inherit: Same as input  ParamDataTypeStr=Inherit: Same as input
  omega_ref : Step  Time=time_init  After=omega_ref_if_pu  SampleTime=0
  id_if_pu : Outport
  iq_if_pu : Outport  Port=2
  tag scope: theta_ref_if_control=global
  wires:
  Unit Delay4/1 -> Sum1/2
  kp/1 -> Sum1/1
  Constant/1 -> iq_if_pu/1
  Sum1/1 -> bounder2/1(u)
  bounder2/1(y) -> [theta_ref_if_control], Unit Delay4/1
  filter_pt1/1(output) -> id_if_pu/1
  id_ref/1 -> filter_pt1/1(input)
  filter_pt2/1(output) -> kp/1
  omega_ref/1 -> filter_pt2/1(input)

== system powertrain_model/driver control/speed_loop ==
  1/Ti : Gain  Gain=-1  SaturateOnIntegerOverflow=on  OutDataTypeStr=Inherit: Same as input  ParamDataTypeStr=Inherit: Same as input
  Constant : Constant  Value=0
  Constant1 : Constant
  Speed control : Subsystem
  iq_ref : Outport
  id_ref : Outport  Port=2
  wires:
  Constant1/1 -> Speed control/2(Speed ref)
  [omega_pu_hat] -> Speed control/1(Rotor speed)
  Speed control/1(torque_ref) -> id_ref/1, 1/Ti/1
  1/Ti/1 -> iq_ref/1

== system powertrain_model/driver control/torque_reference_generator ==
  Rate Limiter : RateLimiter  Commented=through  RisingSlewLimit=0.25  FallingSlewLimit=-0.25  SampleTimeMode=inherited
  Rate Limiter1 : RateLimiter  Commented=through  RisingSlewLimit=0.25  FallingSlewLimit=-0.25  SampleTimeMode=inherited
  Step1 : Step  Time=time_init  After=torque_ref*sin(angle_error)  SampleTime=0
  Step2 : Step  Commented=on  Time=time_init*4  After=-torque_ref  SampleTime=0
  Step3 : Step  Commented=on  Time=0.75  After=-torque_ref*cos(angle_error)*3/2  SampleTime=0
  Step4 : Step  Time=time_init  After=torque_ref*cos(angle_error)  SampleTime=0
  Step5 : Step  Commented=on  Time=0.85  After=torque_ref*cos(angle_error)/2  SampleTime=0
  Sum : Sum  Inputs=++|
  Sum1 : Sum  Inputs=|++
  Sum2 : Sum  Inputs=|++
  reference_d_flt : Subsystem
  reference_q_flt : Subsystem
  iq_ref : Outport
  id_ref : Outport  Port=2
  wires:
  reference_d_flt/1(output) -> id_ref/1
  Step1/1 -> Sum/2
  Step2/1 -> Sum/1
  Step4/1 -> Sum1/1
  Step3/1 -> Sum1/2
  reference_q_flt/1(output) -> iq_ref/1
  Sum/1 -> Rate Limiter/1
  Rate Limiter/1 -> reference_d_flt/1(input)
  Rate Limiter1/1 -> reference_q_flt/1(input)
  Sum1/1 -> Sum2/1
  Sum2/1 -> Rate Limiter1/1
  Step5/1 -> Sum2/2

== system powertrain_model/inverter/Gyro based inverter ==
  uab : Inport
  Demux : Demux  Outputs=2
  Electrical Reference1 : fl_lib/Electrical/Electrical Elements/Electrical Reference
  gyro1 : Subsystem
  gyro2 : Subsystem
  gyro3 : Subsystem
  uvw2alphabeta : MATLAB Function  TreatAsAtomicUnit=on  SystemSampleTime=ts_inv
  u : PMIOPort  Side=Left
  v : PMIOPort  Port=2  Side=Left
  w : PMIOPort  Port=3  Side=Left
  UDC(+) : PMIOPort  Port=4  Side=Right
  UDC(-) : PMIOPort  Port=5  Side=Right
  tag scope: uu_motor=global, uv_motor=global, uw_motor=global
  wires:
  uvw2alphabeta/1(u) -> [uu_motor], [mu]  "mu"
  uvw2alphabeta/2(v) -> [uv_motor], [mv]  "mv"
  uvw2alphabeta/3(w) -> [uw_motor], [mw]  "mw"
  [mu] -> gyro1/1(m)
  [mv] -> gyro2/1(m)
  [mw] -> gyro3/1(m)
  uab/1 -> Demux/1
  Demux/1 -> uvw2alphabeta/1(alpha)
  Demux/2 -> uvw2alphabeta/2(beta)
  connections:
  u/RConn1 -- gyro1/RConn1
  UDC(+)/RConn1 -- gyro3/LConn1 -- gyro2/LConn1 -- gyro1/LConn1
  UDC(-)/RConn1 -- gyro3/LConn2 -- gyro2/LConn2 -- gyro1/LConn2
  gyro2/RConn1 -- v/RConn1
  gyro3/RConn1 -- w/RConn1
  gyro1/RConn2 -- gyro3/RConn2 -- gyro2/RConn2 -- Electrical Reference1/LConn1
